simulink model "ddc"  (R2026a)
settings: Solver=VariableStepAuto
libraries: dsphdlfiltering2 x9, dspmlti4 x1
settings Model: Creator=taokhe  LastModifiedBy=taokhe

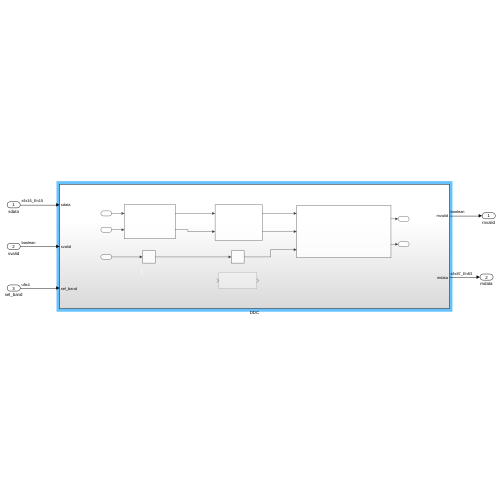
[thumbnail: Simulink's stored preview of the top-level diagram]
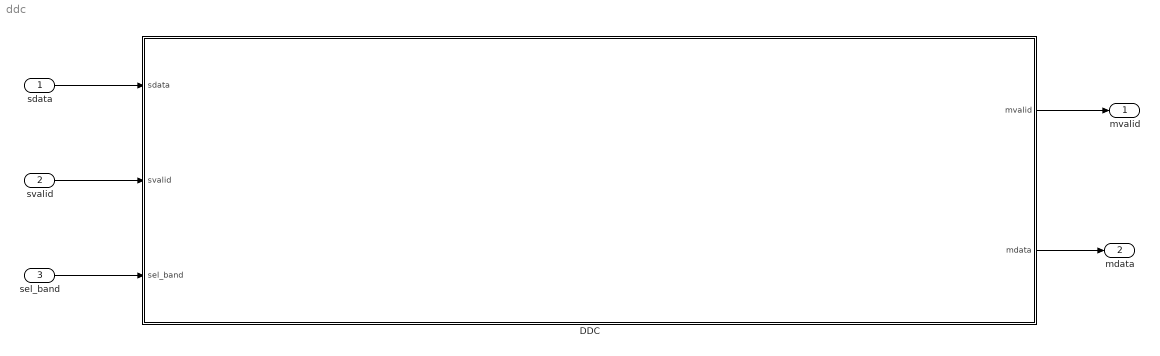
== system ddc ==
  sdata : Inport  OutDataTypeStr=fixdt(1,16,15)
  svalid : Inport  Port=2  OutDataTypeStr=boolean
  sel_band : Inport  Port=3  OutDataTypeStr=fixdt(0,4,0)
  DDC : Subsystem
  mvalid : Outport
  mdata : Outport  Port=2
  wires:
  sdata/1 -> DDC/1(sdata)
  svalid/1 -> DDC/2(svalid)
  sel_band/1 -> DDC/3(sel_band)
  DDC/1(mvalid) -> mvalid/1
  DDC/2(mdata) -> mdata/1

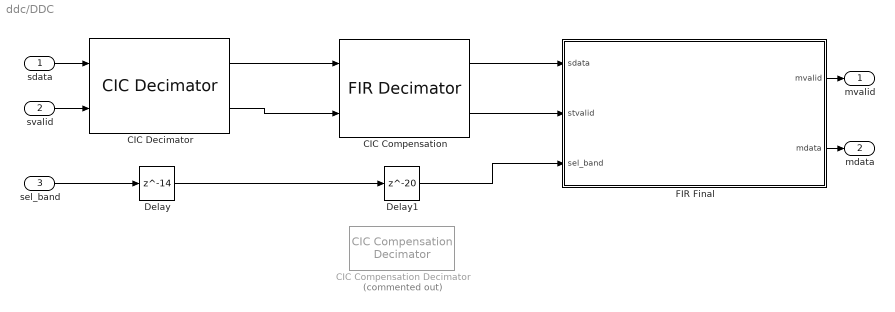
== system ddc/DDC ==
  sdata : Inport
  svalid : Inport  Port=2
  sel_band : Inport  Port=3
  CIC Compensation : dsphdlfiltering2/FIR Decimator  NumeratorSource=Property  Numerator=[1.2452656025148105e-18 0.001600652863930364 0.0013174534552817744 -0.001869217448560894 -0.0043336136492038557 3.9411829952775998e-18 0.0084623903178864569 0.0070770504736392308 -0.0094027236100340285 -0.019932921419138615 9.9988543901227614e-18 0.033512266120542422 0.026943639374828902 -0.035607242376925904 -0.078759811193972379 1.4856729672754624e-17 0.198132880044913 0.37285919704681353 0.37285919704681353 0.198132880044913 1.4856729672754624e-17 -0.078759811193972379 -0.035607242376925904 0.026943639374828902 0.033512266120542422 9.9988543901227614e-18 -0.019932921419138615 -0.0094027236100340285 0.0070770504736392308 0.0084623903178864569 3.9411829952775998e-18 -0.0043336136492038557 -0.001869217448560894 0.0013174534552817744 0.001600652863930364 1.2452656025148105e-18]  NumeratorPrototype=[]  FilterStructure=Direct form systolic  DecimationFactor=2  NumCycles=1  OptimizeSymmCoeff=on  SimulateUsing=Code generation  roundingMode=Floor  overflowMode=off  CoefficientsDataTypeStr=Inherit: Same word length as input  ResetInputPort=off  HDLGlobalReset=off
  CIC Compensation Decimator : dspmlti4/CIC Compensation Decimator  Commented=on  CICRateChangeFactor=5  CICNumSections=2  CICDifferentialDelay=1  DecimationFactor=1  DesignForMinimumOrder=on  FilterOrder=12  PassbandFrequency=40e6  StopbandFrequency=100e6  PassbandRipple=0.01  StopbandAttenuation=120  SampleRateMode=Specify on dialog  SampleRate=250e6  AllowArbitraryInputLength=off  SimulateUsing=Interpreted execution  roundingMode=Floor  coeffsDataTypeStr=fixdt(1,16)
  CIC Decimator : dsphdlfiltering2/CIC Decimator  DecimationSource=Property  DecimationFactor=5  MaxDecimationFactor=2  DifferentialDelay=1  NumSections=2  GainCorrection=on  SimulateUsing=Code generation  OutputDataType=Full precision  OutputWordLength=16  ResetInputPort=off  HDLGlobalReset=off
  Delay : Delay  DelayLength=14
  Delay1 : Delay  DelayLength=20
  FIR Final : Subsystem
  mvalid : Outport
  mdata : Outport  Port=2
  wires:
  CIC Decimator/1 -> CIC Compensation/1
  CIC Decimator/2 -> CIC Compensation/2
  CIC Compensation/1 -> FIR Final/1(sdata)
  CIC Compensation/2 -> FIR Final/2(stvalid)
  FIR Final/2(mdata) -> mdata/1
  svalid/1 -> CIC Decimator/2
  FIR Final/1(mvalid) -> mvalid/1
  sel_band/1 -> Delay/1
  sdata/1 -> CIC Decimator/1
  Delay/1 -> Delay1/1
  Delay1/1 -> FIR Final/3(sel_band)

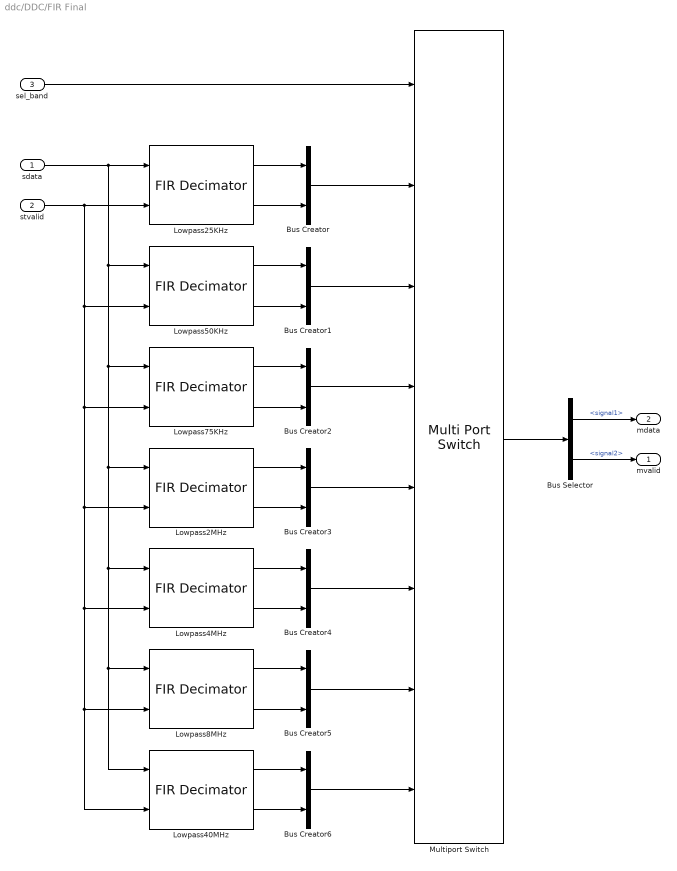
== system ddc/DDC/FIR Final ==
  sdata : Inport
  stvalid : Inport  Port=2
  sel_band : Inport  Port=3
  Bus Creator{,1..6} (7 alike) : BusCreator  Inputs=2
  Bus Selector : BusSelector  OutputSignals=signal1,signal2
  Lowpass25KHz : dsphdlfiltering2/FIR Decimator  NumeratorSource=Property  Numerator=[1.2452656025148105e-18 0.001600652863930364 0.0013174534552817744 -0.001869217448560894 -0.0043336136492038557 3.9411829952775998e-18 0.0084623903178864569 0.0070770504736392308 -0.0094027236100340285 -0.019932921419138615 9.9988543901227614e-18 0.033512266120542422 0.026943639374828902 -0.035607242376925904 -0.078759811193972379 1.4856729672754624e-17 0.198132880044913 0.37285919704681353 0.37285919704681353 0.198132880044913 1.4856729672754624e-17 -0.078759811193972379 -0.035607242376925904 0.026943639374828902 0.033512266120542422 9.9988543901227614e-18 -0.019932921419138615 -0.0094027236100340285 0.0070770504736392308 0.0084623903178864569 3.9411829952775998e-18 -0.0043336136492038557 -0.001869217448560894 0.0013174534552817744 0.001600652863930364 1.2452656025148105e-18]  NumeratorPrototype=[]  FilterStructure=Direct form systolic  DecimationFactor=2  NumCycles=1  OptimizeSymmCoeff=on  SimulateUsing=Code generation  roundingMode=Floor  overflowMode=off  CoefficientsDataTypeStr=Inherit: Same word length as input  ResetInputPort=off  HDLGlobalReset=off
  Lowpass2MHz : dsphdlfiltering2/FIR Decimator  NumeratorSource=Property  Numerator=[1.2452656025148105e-18 0.001600652863930364 0.0013174534552817744 -0.001869217448560894 -0.0043336136492038557 3.9411829952775998e-18 0.0084623903178864569 0.0070770504736392308 -0.0094027236100340285 -0.019932921419138615 9.9988543901227614e-18 0.033512266120542422 0.026943639374828902 -0.035607242376925904 -0.078759811193972379 1.4856729672754624e-17 0.198132880044913 0.37285919704681353 0.37285919704681353 0.198132880044913 1.4856729672754624e-17 -0.078759811193972379 -0.035607242376925904 0.026943639374828902 0.033512266120542422 9.9988543901227614e-18 -0.019932921419138615 -0.0094027236100340285 0.0070770504736392308 0.0084623903178864569 3.9411829952775998e-18 -0.0043336136492038557 -0.001869217448560894 0.0013174534552817744 0.001600652863930364 1.2452656025148105e-18]  NumeratorPrototype=[]  FilterStructure=Direct form systolic  DecimationFactor=2  NumCycles=1  OptimizeSymmCoeff=on  SimulateUsing=Code generation  roundingMode=Floor  overflowMode=off  CoefficientsDataTypeStr=Inherit: Same word length as input  ResetInputPort=off  HDLGlobalReset=off
  Lowpass40MHz : dsphdlfiltering2/FIR Decimator  NumeratorSource=Property  Numerator=[1.2452656025148105e-18 0.001600652863930364 0.0013174534552817744 -0.001869217448560894 -0.0043336136492038557 3.9411829952775998e-18 0.0084623903178864569 0.0070770504736392308 -0.0094027236100340285 -0.019932921419138615 9.9988543901227614e-18 0.033512266120542422 0.026943639374828902 -0.035607242376925904 -0.078759811193972379 1.4856729672754624e-17 0.198132880044913 0.37285919704681353 0.37285919704681353 0.198132880044913 1.4856729672754624e-17 -0.078759811193972379 -0.035607242376925904 0.026943639374828902 0.033512266120542422 9.9988543901227614e-18 -0.019932921419138615 -0.0094027236100340285 0.0070770504736392308 0.0084623903178864569 3.9411829952775998e-18 -0.0043336136492038557 -0.001869217448560894 0.0013174534552817744 0.001600652863930364 1.2452656025148105e-18]  NumeratorPrototype=[]  FilterStructure=Direct form systolic  DecimationFactor=2  NumCycles=1  OptimizeSymmCoeff=on  SimulateUsing=Code generation  roundingMode=Floor  overflowMode=off  CoefficientsDataTypeStr=Inherit: Same word length as input  ResetInputPort=off  HDLGlobalReset=off
  Lowpass4MHz : dsphdlfiltering2/FIR Decimator  NumeratorSource=Property  Numerator=[1.2452656025148105e-18 0.001600652863930364 0.0013174534552817744 -0.001869217448560894 -0.0043336136492038557 3.9411829952775998e-18 0.0084623903178864569 0.0070770504736392308 -0.0094027236100340285 -0.019932921419138615 9.9988543901227614e-18 0.033512266120542422 0.026943639374828902 -0.035607242376925904 -0.078759811193972379 1.4856729672754624e-17 0.198132880044913 0.37285919704681353 0.37285919704681353 0.198132880044913 1.4856729672754624e-17 -0.078759811193972379 -0.035607242376925904 0.026943639374828902 0.033512266120542422 9.9988543901227614e-18 -0.019932921419138615 -0.0094027236100340285 0.0070770504736392308 0.0084623903178864569 3.9411829952775998e-18 -0.0043336136492038557 -0.001869217448560894 0.0013174534552817744 0.001600652863930364 1.2452656025148105e-18]  NumeratorPrototype=[]  FilterStructure=Direct form systolic  DecimationFactor=2  NumCycles=1  OptimizeSymmCoeff=on  SimulateUsing=Code generation  roundingMode=Floor  overflowMode=off  CoefficientsDataTypeStr=Inherit: Same word length as input  ResetInputPort=off  HDLGlobalReset=off
  Lowpass50KHz : dsphdlfiltering2/FIR Decimator  NumeratorSource=Property  Numerator=[1.2452656025148105e-18 0.001600652863930364 0.0013174534552817744 -0.001869217448560894 -0.0043336136492038557 3.9411829952775998e-18 0.0084623903178864569 0.0070770504736392308 -0.0094027236100340285 -0.019932921419138615 9.9988543901227614e-18 0.033512266120542422 0.026943639374828902 -0.035607242376925904 -0.078759811193972379 1.4856729672754624e-17 0.198132880044913 0.37285919704681353 0.37285919704681353 0.198132880044913 1.4856729672754624e-17 -0.078759811193972379 -0.035607242376925904 0.026943639374828902 0.033512266120542422 9.9988543901227614e-18 -0.019932921419138615 -0.0094027236100340285 0.0070770504736392308 0.0084623903178864569 3.9411829952775998e-18 -0.0043336136492038557 -0.001869217448560894 0.0013174534552817744 0.001600652863930364 1.2452656025148105e-18]  NumeratorPrototype=[]  FilterStructure=Direct form systolic  DecimationFactor=2  NumCycles=1  OptimizeSymmCoeff=on  SimulateUsing=Code generation  roundingMode=Floor  overflowMode=off  CoefficientsDataTypeStr=Inherit: Same word length as input  ResetInputPort=off  HDLGlobalReset=off
  Lowpass75KHz : dsphdlfiltering2/FIR Decimator  NumeratorSource=Property  Numerator=[1.2452656025148105e-18 0.001600652863930364 0.0013174534552817744 -0.001869217448560894 -0.0043336136492038557 3.9411829952775998e-18 0.0084623903178864569 0.0070770504736392308 -0.0094027236100340285 -0.019932921419138615 9.9988543901227614e-18 0.033512266120542422 0.026943639374828902 -0.035607242376925904 -0.078759811193972379 1.4856729672754624e-17 0.198132880044913 0.37285919704681353 0.37285919704681353 0.198132880044913 1.4856729672754624e-17 -0.078759811193972379 -0.035607242376925904 0.026943639374828902 0.033512266120542422 9.9988543901227614e-18 -0.019932921419138615 -0.0094027236100340285 0.0070770504736392308 0.0084623903178864569 3.9411829952775998e-18 -0.0043336136492038557 -0.001869217448560894 0.0013174534552817744 0.001600652863930364 1.2452656025148105e-18]  NumeratorPrototype=[]  FilterStructure=Direct form systolic  DecimationFactor=2  NumCycles=1  OptimizeSymmCoeff=on  SimulateUsing=Code generation  roundingMode=Floor  overflowMode=off  CoefficientsDataTypeStr=Inherit: Same word length as input  ResetInputPort=off  HDLGlobalReset=off
  Lowpass8MHz : dsphdlfiltering2/FIR Decimator  NumeratorSource=Property  Numerator=[1.2452656025148105e-18 0.001600652863930364 0.0013174534552817744 -0.001869217448560894 -0.0043336136492038557 3.9411829952775998e-18 0.0084623903178864569 0.0070770504736392308 -0.0094027236100340285 -0.019932921419138615 9.9988543901227614e-18 0.033512266120542422 0.026943639374828902 -0.035607242376925904 -0.078759811193972379 1.4856729672754624e-17 0.198132880044913 0.37285919704681353 0.37285919704681353 0.198132880044913 1.4856729672754624e-17 -0.078759811193972379 -0.035607242376925904 0.026943639374828902 0.033512266120542422 9.9988543901227614e-18 -0.019932921419138615 -0.0094027236100340285 0.0070770504736392308 0.0084623903178864569 3.9411829952775998e-18 -0.0043336136492038557 -0.001869217448560894 0.0013174534552817744 0.001600652863930364 1.2452656025148105e-18]  NumeratorPrototype=[]  FilterStructure=Direct form systolic  DecimationFactor=2  NumCycles=1  OptimizeSymmCoeff=on  SimulateUsing=Code generation  roundingMode=Floor  overflowMode=off  CoefficientsDataTypeStr=Inherit: Same word length as input  ResetInputPort=off  HDLGlobalReset=off
  Multiport Switch : MultiPortSwitch  Inputs=7  SaturateOnIntegerOverflow=off  InputSameDT=off
  mvalid : Outport
  mdata : Outport  Port=2
  wires:
  sdata/1 -> Lowpass40MHz/1, Lowpass8MHz/1, Lowpass4MHz/1, Lowpass2MHz/1, Lowpass75KHz/1, Lowpass50KHz/1, Lowpass25KHz/1
  stvalid/1 -> Lowpass40MHz/2, Lowpass8MHz/2, Lowpass4MHz/2, Lowpass2MHz/2, Lowpass75KHz/2, Lowpass50KHz/2, Lowpass25KHz/2
  Lowpass25KHz/2 -> Bus Creator/2
  Lowpass25KHz/1 -> Bus Creator/1
  Lowpass50KHz/1 -> Bus Creator1/1
  Lowpass50KHz/2 -> Bus Creator1/2
  Lowpass75KHz/1 -> Bus Creator2/1
  Lowpass75KHz/2 -> Bus Creator2/2
  Lowpass2MHz/1 -> Bus Creator3/1
  Lowpass2MHz/2 -> Bus Creator3/2
  Lowpass4MHz/1 -> Bus Creator4/1
  Lowpass4MHz/2 -> Bus Creator4/2
  Lowpass40MHz/1 -> Bus Creator6/1
  Lowpass40MHz/2 -> Bus Creator6/2
  Lowpass8MHz/1 -> Bus Creator5/1
  Lowpass8MHz/2 -> Bus Creator5/2
  Bus Creator6/1 -> Multiport Switch/8
  Bus Creator5/1 -> Multiport Switch/7
  Bus Creator4/1 -> Multiport Switch/6
  Bus Creator3/1 -> Multiport Switch/5
  Bus Creator2/1 -> Multiport Switch/4
  Bus Creator1/1 -> Multiport Switch/3
  Bus Creator/1 -> Multiport Switch/2
  sel_band/1 -> Multiport Switch/1
  Multiport Switch/1 -> Bus Selector/1
  Bus Selector/2 -> mvalid/1  "<signal2>"
  Bus Selector/1 -> mdata/1  "<signal1>"
